simulink model "turbo_controller"  (R2025a)
settings: Solver=FixedStepAuto  StartTime=0.0  StopTime=inf  FixedStep=0.001  RelTol=1e-3
PostLoadFcn:
  | % 自动定位同目录CubeMX文件；不需要外部初始化脚本。
  | codertarget.data.setParameterValue('turbo_controller','STM32CubeMX.ProjectFile',fullfile(fileparts(get_param('turbo_controller','FileName')),'turbo_f407.ioc'));
InitFcn:
  | % 中文说明：按原控制器字段与类型创建三组接口总线；控制参数已内嵌。
  | tc_names=["EValve_Cycle" "EValve_Open" "Eblast_Cycle" "Eblast_Open" "Motor_Cycle" "Motor_Open" "EValve_Enable" "Eblast_Enable" "Motor_Enable" "SWO_Firework" "SWO_BleedAir" "EngineState" "Flag_ECUReset_Clear" "Flag_ECUReset_Save" "Flag_Reset_Enable" "Accelerator" "Nc_dem" "Nc"]; tc_types=["uint16" "uint16" "uint16" "uint16" "uint16" "uint16" "uint8" "uint8" "uint8" "uint8" "uint8" "uint8" "uint8" "uint8" "uint8" "single" "single" "single"];
  | for tc_k=1:numel(tc_names)
  |  tc_e(tc_k)=Simulink.BusElement; tc_e(tc_k).Name=char(tc_names(tc_k)); tc_e(tc_k).DataType=char(tc_types(tc_k));
  | end
  | EngineControl_Out=Simulink.Bus; EngineControl_Out.DataScope='Exported'; EngineControl_Out.Elements=tc_e;
  | clear tc_e tc_names tc_types tc_k
  | tc_names=["savedata1" "savedata2" "savedata3" "savedata4" "savedata5" "savedata6" "savedata7" "savedata8" "savedata9" "savedata10" "savedata11" "savedata12" "savedata13" "savedata14" "savedata15" "savedata16" "savedata17" "savedata18" "savedata19" "savedata20" "savedata21" "savedata22" "savedata23" "savedata24" "savedata25"]; tc_types=["single" "single" "single" "single" "single" "single" "single" "single" "single" "single" "single" "single" "single" "single" "single" "single" "single" "single" "single" "single" "single" "single" "single" "single" "single"];
  | for tc_k=1:numel(tc_names)
  |  tc_e(tc_k)=Simulink.BusElement; tc_e(tc_k).Name=char(tc_names(tc_k)); tc_e(tc_k).DataType=char(tc_types(tc_k));
  | end
  | SaveData_Out=Simulink.Bus; SaveData_Out.DataScope='Exported'; SaveData_Out.Elements=tc_e;
  | clear tc_e tc_names tc_types tc_k
  | tc_names=["senddata1" "senddata2" "senddata3" "senddata4" "senddata5" "senddata6" "senddata7" "senddata8" "senddata9" "senddata10" "senddata11" "senddata12" "senddata13" "senddata14" "senddata15" "senddata16" "senddata17" "senddata18" "senddata19" "senddata20" "senddata21" "senddata22" "senddata23" "senddata24" "senddata25" "senddata26" "senddata27" "senddata28" "senddata29"]; tc_types=["uint8" "uint8" "uint8" "uint8" "uint8" "uint8" "uint8" "uint8" "uint8" "uint8" "uint8" "uint8" "uint8" "uint8" "uint8" "uint8" "uint8" "uint8" "uint8" "uint8" "uint8" "uint8" "uint8" "uint8" "uint8" "uint8" "uint8" "uint8" "uint8"];
  | for tc_k=1:numel(tc_names)
  |  tc_e(tc_k)=Simulink.BusElement; tc_e(tc_k).Name=char(tc_names(tc_k)); tc_e(tc_k).DataType=char(tc_types(tc_k));
  | end
  | SendData_Out=Simulink.Bus; SendData_Out.DataScope='Exported'; SendData_Out.Elements=tc_e;
  | clear tc_e tc_names tc_types tc_k
  | 
  | % 以下为接口中文说明；只设置描述，不改变数值或数据类型。
  | EngineControl_Out.Description='执行控制输出（阀、电机、点火、状态及复位请求）';
  | tc_cn=["EValve_Cycle（主油阀周期计数（每计数2毫秒））" "EValve_Open（主油阀开通计数（每计数2毫秒））" "Eblast_Cycle（副油阀周期计数（每计数2毫秒））" "Eblast_Open（副油阀开通计数（每计数2毫秒））" "Motor_Cycle（起动电机周期计数）" "Motor_Open（起动电机开通计数）" "EValve_Enable（主油阀驱动使能）" "Eblast_Enable（副油阀驱动使能）" "Motor_Enable（起动电机使能）" "SWO_Firework（点火器使能（1开））" "SWO_BleedAir（引气阀使能（1开））" "EngineState（发动机状态）" "Flag_ECUReset_Clear（清除复位恢复状态请求）" "Flag_ECUReset_Save（保存复位恢复数据请求）" "Flag_Reset_Enable（处理器软件复位请求）" "Accelerator（油门／油泵给定控制量）" "Nc_dem（控制目标转速）" "Nc（发动机反馈转速（转每分））"];
  | tc_elements=EngineControl_Out.Elements;
  | for tc_k=1:numel(tc_cn)
  |  tc_elements(tc_k).Description=char(tc_cn(tc_k));
  | end
  | EngineControl_Out.Elements=tc_elements;
  | clear tc_cn tc_elements tc_k
  | SaveData_Out.Description='25项运行记录；字段含义按当前模型数据来源解释';
  | tc_cn=["savedata1（指令回显记录）" "savedata2（入口总温记录（℃））" "savedata3（电源电压记录）" "savedata4（排气温度记录（℃））" "savedata5（标定燃油压力记录）" "savedata6（副油阀占空比记录（％））" "savedata7（主油阀占空比记录（％））" "savedata8（温度修正转速记录）" "savedata9（开关输出及反馈位域）" "savedata10（物理转速记录）" "savedata11（油泵目标给定原始值）" "savedata12（起动电机占空比记录（％））" "savedata13（发动机状态码记录）" "savedata14（故障告警位域记录）" "savedata15（模型记录帧序号）" "savedata16（处理器温度记录（℃））" "savedata17（装订转速记录（沿用旧电源字段名））" "savedata18（导航高度记录）" "savedata19（飞行空速记录）" "savedata20（主阀旧记录位（恒零保留））" "savedata21（第21项保留记录（恒零））" "savedata22（保留记录项22）" "savedata23（保留记录项23）" "savedata24（保留记录项24）" "savedata25（保留记录项25）"];
  | tc_elements=SaveData_Out.Elements;
  | for tc_k=1:numel(tc_cn)
  |  tc_elements(tc_k).Description=char(tc_cn(tc_k));
  | end
  | SaveData_Out.Elements=tc_elements;
  | clear tc_cn tc_elements tc_k
  | SendData_Out.Description='29字段回传及外设命令接口；板端上位机帧只取第3至27字段';
  | tc_cn=["senddata1（回传发送允许标志（不直接上线路））" "senddata2（回传载荷长度25字节）" "senddata3（回传指令回显字节）" "senddata4（总温编码字节（℃＋80））" "senddata5（电源电压编码字节）" "senddata6（排温编码高字节）" "senddata7（排温编码低字节）" "senddata8（燃油压力编码高字节）" "senddata9（燃油压力编码低字节）" "senddata10（副油阀占空比字节（％））" "senddata11（主油阀占空比字节（％））" "senddata12（修正转速编码高字节）" "senddata13（修正转速编码低字节）" "senddata14（驱动及反馈状态位域）" "senddata15（物理转速编码高字节）" "senddata16（物理转速编码低字节）" "senddata17（油泵目标给定高字节（串口二使用））" "senddata18（油泵目标给定低字节（串口二使用））" "senddata19（起动电机占空比命令（串口一使用））" "senddata20（发动机状态码字节）" "senddata21（故障告警位域字节）" "senddata22（帧序号占位（板端另行填写））" "senddata23（处理器温度编码（℃＋50））" "senddata24（控制目标转速编码高字节）" "senddata25（控制目标转速编码低字节）" "senddata26（占位字节（板端改填实测泵速高字节））" "senddata27（占位字节（板端改填实测泵速低字节））" "senddata28（装订转速高字节（本板未发送））" "senddata29（装订转速低字节（本板未发送））"];
  | tc_elements=SendData_Out.Elements;
  | for tc_k=1:numel(tc_cn)
  |  tc_elements(tc_k).Description=char(tc_cn(tc_k));
  | end
  | SendData_Out.Elements=tc_elements;
  | clear tc_cn tc_elements tc_k
  | 
  | 
  | % FRAM模块化事务：接口类型和上电初始状态，随模型保存，无外部初始化文件。
  | clear FM_elements
  | FM_elements(1)=Simulink.BusElement;FM_elements(1).Name='phase';FM_elements(1).DataType='uint8';FM_elements(1).Dimensions=[1 1];FM_elements(1).Description='phase（当前事务阶段）';
  | FM_elements(2)=Simulink.BusElement;FM_elements(2).Name='a';FM_elements(2).DataType='uint8';FM_elements(2).Dimensions=[64 1];FM_elements(2).Description='a（启动时缓存的首区64字节）';
  | FM_elements(3)=Simulink.BusElement;FM_elements(3).Name='active';FM_elements(3).DataType='uint16';FM_elements(3).Dimensions=[1 1];FM_elements(3).Description='active（当前有效记录区地址）';
  | FM_elements(4)=Simulink.BusElement;FM_elements(4).Name='generation';FM_elements(4).DataType='uint32';FM_elements(4).Dimensions=[1 1];FM_elements(4).Description='generation（当前有效记录代号）';
  | FM_elements(5)=Simulink.BusElement;FM_elements(5).Name='record';FM_elements(5).DataType='uint8';FM_elements(5).Dimensions=[64 1];FM_elements(5).Description='record（本次冻结的待写记录）';
  | FM_elements(6)=Simulink.BusElement;FM_elements(6).Name='addr';FM_elements(6).DataType='uint16';FM_elements(6).Dimensions=[1 1];FM_elements(6).Description='addr（本次备用写入地址）';
  | FM_elements(7)=Simulink.BusElement;FM_elements(7).Name='lastSave';FM_elements(7).DataType='single';FM_elements(7).Dimensions=[1 1];FM_elements(7).Description='lastSave（上次开始保存的秒数）';
  | FM_elements(8)=Simulink.BusElement;FM_elements(8).Name='lastState';FM_elements(8).DataType='uint8';FM_elements(8).Dimensions=[1 1];FM_elements(8).Description='lastState（上次保存时的发动机状态）';
  | FM_elements(9)=Simulink.BusElement;FM_elements(9).Name='boot';FM_elements(9).DataType='boolean';FM_elements(9).Dimensions=[1 1];FM_elements(9).Description='boot（启动记录是否允许恢复）';
  | FM_elements(10)=Simulink.BusElement;FM_elements(10).Name='consumed';FM_elements(10).DataType='boolean';FM_elements(10).Dimensions=[1 1];FM_elements(10).Description='consumed（本次启动恢复通知是否已发送）';
  | FM_elements(11)=Simulink.BusElement;FM_elements(11).Name='payload';FM_elements(11).DataType='uint8';FM_elements(11).Dimensions=[20 1];FM_elements(11).Description='payload（当前20字节恢复内容）';
  | ... (+35 lines)
model workspace (MAT data in the model file):
  CRC16_Table_Reference = [0 4129 8258 12387 16516 20645 24774 28903 33032 37161 41290 45419 ... (256 elements, 256x1)]
  PE_Kaer = [0.15402 0.15402 0.12264 0.10076 0.09481 0.07601 0.07111 0.0569 0.05198 0.04926 0.05308 0.04325 ... (13 elements, 1x13)]
  PE_Nr = [21.2982 61.4260372 67.7475458 72.7394382 76.845934 80.6988798 83.8449282 86.6491912 88.9382406 89.178606 91.1938214 93.4068058 ... (13 elements, 1x13)]
  PE_Pump_Translate = 33.5999984741
  PE_RotaSpeed_Translate = 860
  PE_Taer = [0.4939154 0.4939154 0.40780982 0.34066978 0.31622756 0.30405716 0.34300244 0.26785022 0.37393554 0.23914836 0.44563948 0.31044662 ... (13 elements, 1x13)]
  PF_ACCFULLRANGE = 3360
  PF_Flag_ECUReset = 0
  PF_Flag_rx_suc = 1
  PF_Gear_Info = [40000; 45000; 50000; 55000; 57000; 59000; 60000; 61000; 61000; 61000; 61000; 61000]
  PF_K_TiaoJie = 1
  PF_Kpu = 10
  PF_MySet_Rxdata = [0 0 0 0 0 0 0 0 0 0 0 0 ... (50 elements, 50x1)]
  PF_MyUsart1_Rxdata = [0 0 0 0 0 0 0 0 0 0 0 0 ... (50 elements, 50x1)]
  PF_MyUsart2_Rxdata = [0 0 0 0 0 0 0 0 0 0 0 0 ... (50 elements, 50x1)]
  PF_Reset_Information = [0 0 0 0 0 0 0 0 0 0 0 0 ... (20 elements, 20x1)]
  PF_Sensor_X1_T4 = [0 4095]
  PF_Sensor_X2_T4 = [0 1.66666698456]
  PF_Sensor_X3_T4 = [0 504 999 1497 2010 2529 3051 3568 4076 4571 4959]
  PF_Sensor_X_P2 = [0.5 3]
  PF_Sensor_X_Poil = [0.5 3]
  PF_Sensor_X_T1t = [-50 300]
  PF_Sensor_X_Vpower = [0 3]
  PF_Sensor_X_Vpump = [0 3]
  PF_Sensor_Y1_T4 = [0 3]
  PF_Sensor_Y2_T4 = [0 5000]
  PF_Sensor_Y3_T4 = [0 100 200 300 400 500 600 700 800 900 980]
  PF_Sensor_Y_P2 = [0 1000]
  PF_Sensor_Y_Poil = [0 1000]
  PF_Sensor_Y_T1t = [-50 300]
  PF_Sensor_Y_Vpower = [0 33]
  PF_Sensor_Y_Vpump = [0 33]
  PG_CtrlMode_CloseLoop : mpt.Parameter (value not decoded)
  PG_CtrlMode_ManualAcc : mpt.Parameter (value not decoded)
  PG_CtrlMode_Origin : mpt.Parameter (value not decoded)
  PG_CtrlMode_Start : mpt.Parameter (value not decoded)
  PG_CtrlMode_Stop : mpt.Parameter (value not decoded)
  PG_ES_Clp : mpt.Parameter (value not decoded)
  PG_ES_EngStart : mpt.Parameter (value not decoded)
  PG_ES_Manual : mpt.Parameter (value not decoded)
  PG_ES_Origin : mpt.Parameter (value not decoded)
  PG_ES_Stop : mpt.Parameter (value not decoded)
  PG_Instr_BleedAirSet : mpt.Parameter (value not decoded)
  PG_Instr_CloseLoop : mpt.Parameter (value not decoded)
  PG_Instr_ECUReSet : mpt.Parameter (value not decoded)
  PG_Instr_EValveSet : mpt.Parameter (value not decoded)
  PG_Instr_EblastSet : mpt.Parameter (value not decoded)
  PG_Instr_Erase : mpt.Parameter (value not decoded)
  PG_Instr_FireWorkSet : mpt.Parameter (value not decoded)
  PG_Instr_ManualPlus : mpt.Parameter (value not decoded)
  PG_Instr_ManualrReduce : mpt.Parameter (value not decoded)
  PG_Instr_MotorSet : mpt.Parameter (value not decoded)
  PG_Instr_OilSet : mpt.Parameter (value not decoded)
  PG_Instr_SelfCheck : mpt.Parameter (value not decoded)
  PG_Instr_Start : mpt.Parameter (value not decoded)
  PG_Instr_Stop : mpt.Parameter (value not decoded)
  PG_Instr_StopZero : Simulink.Parameter (value not decoded)
  PG_Location_Air : Simulink.Parameter (value not decoded)
  PG_Location_Gnd : Simulink.Parameter (value not decoded)
  PG_ServoCtrlMode_CloseLoop : Simulink.Parameter (value not decoded)
  PG_ServoCtrlMode_CloseLoopMax : Simulink.Parameter (value not decoded)
  PG_ServoCtrlMode_CloseLoopMin : Simulink.Parameter (value not decoded)
  PG_ServoCtrlMode_ManualAcc : Simulink.Parameter (value not decoded)
  PG_ServoCtrlMode_ManualAccMax : Simulink.Parameter (value not decoded)
  PG_ServoCtrlMode_ManualAccMin : Simulink.Parameter (value not decoded)
  PG_SpeedDot_Permit : Simulink.Parameter (value not decoded)
  PL_EngineModel_Actuator = [0 10 100]
  PL_EngineModel_EngineStar_Press_P2 = [1013 1098.4 1099.144828 1099.931034 1103.613793 1162.662069 1143.793103 1131.006897 1123.186207 1117.6 1114 1111.806897 ... (127 elements, 1x127)]
  PL_EngineModel_EngineStar_RotaSpeed = [200 2000 9584 9660 10220 10240 10260 10288 10308 10368 10380 10408 ... (127 elements, 1x127)]
  PL_EngineModel_EngineStar_Temp_Exhaust = [128 129 129.1 130 131 131.1 132 133 134 134.1 135 135.1 ... (127 elements, 1x127)]
  PL_EngineModel_EngineStar_Time = [0.05 0.1 0.15 0.2 0.25 0.3 0.35 0.4 0.45 0.5 0.55 0.6 ... (127 elements, 1x127)]
  PL_EngineModel_IdleAbove_Nr = [0 21.2982 61.4260372 67.7475458 72.7394382 76.845934 80.6988798 83.8449282 86.6491912 88.9382406 89.178606 91.1938214 ... (14 elements, 1x14)]
  PL_EngineModel_IdleAbove_P2r = [0.986923266716 1.57907722675 1.81593881076 1.99358499877 2.23044658278 2.43770046879 2.65482358747 2.84233900814 3.03972366149 3.18776215149 3.25684678016 3.3950160375 ... (14 elements, 1x14)]
  PL_EngineModel_IdleAbove_Tempr = [0.0536001429337 1.07200285867 1.63301768805 1.63659103091 1.66875111667 1.72592460247 1.77595140254 1.86171163123 1.95461854565 2.03323208862 2.03323208862 2.13685903162 ... (14 elements, 1x14)]
  PL_EngineModel_IdleAbove_Ter = [0.42434128 0.42434128 0.42434128 0.30669408 0.23570008 0.22150128 0.1997974 0.23803274 0.16115638 0.24279948 0.13600422 0.31308354 ... (14 elements, 1x14)]
  PL_EngineModel_IdleAbove_Wfr = [0 10.142 23.8337 27.8905 31.9473 36.0041 40.0609 44.1177 48.1745 52.2313 52.7384 56.7952 ... (14 elements, 1x14)]
  PL_EngineModel_Press_P2 = [400 400 400 400 400 400 400 400 400 400]
  PL_EngineModel_Rotaspeed = [0 20000 96400]
  PL_EngineModel_Temp_Exhaust = [500 500 500 500 500 500 500 500 500 500]
  PL_Kaer = [0.1 0.1 0.1 0.1 0.1 0.1]
  PL_Nr = [50 60 70 80 90 100]
  PL_Taer = [0.1 0.1 0.1 0.1 0.1 0.1]
  Sig : Simulink.Signal (value not decoded)
  Ts_ms : Simulink.Parameter (value not decoded)
  false : Simulink.Parameter (value not decoded)
  true : Simulink.Parameter (value not decoded)
symbols that are objects in the model workspace (value not decoded): PG_CtrlMode_CloseLoop, PG_CtrlMode_ManualAcc, PG_CtrlMode_Origin, PG_CtrlMode_Start, PG_CtrlMode_Stop, PG_ES_Clp, PG_ES_EngStart, PG_ES_Manual, PG_ES_Origin, PG_ES_Stop, PG_Instr_BleedAirSet, PG_Instr_CloseLoop, PG_Instr_EblastSet, PG_Instr_ECUReSet, PG_Instr_Erase, PG_Instr_EValveSet, PG_Instr_FireWorkSet, PG_Instr_ManualPlus, PG_Instr_ManualrReduce, PG_Instr_MotorSet, PG_Instr_OilSet, PG_Instr_SelfCheck, PG_Instr_Start, PG_Instr_Stop, PG_Instr_StopZero, PG_ServoCtrlMode_CloseLoop, PG_ServoCtrlMode_CloseLoopMax, PG_ServoCtrlMode_CloseLoopMin, PG_ServoCtrlMode_ManualAcc, PG_ServoCtrlMode_ManualAccMax, PG_ServoCtrlMode_ManualAccMin, Ts_ms
libraries: simulink x97, stm32blockslib x10, stm32f4xxblockslib x8
(part 12 of 26)

== system turbo_controller/BoardOutput_串口封装与阀门时序/Out02_Timing（阀门与点火时序）/MainValve（主阀周期与开度）_719 ==
  note: 主阀怎样按周期形成开启区间
      |
      | 本模块收到使能Enable、周期计数Cycle、开启计数Open，以及父级给出的偶数毫秒节拍Even。它输出
      | 的是逻辑开启状态On，父级随后才按低有效电路把它取反成引脚电平。
      |
      | 先检查Enable是否非零、Cycle是否非零，两者都成立才允许运行。对Cycle为零的情况，SafeCycle提
      | 供1作为取余用的安全分母，但运行许可仍为假，所以不会因为避免除零而误开阀。
      |
      | 内部Phase记住周期位置，在2 ms节拍内按先归一化、后推进的分支更新。位置到周期末尾通过取余回
      | 到起点；位置小于Open时On为真，其余区间为假。
      |
      | 例如Cycle=30、Open=15，约每60 ms重复一次，其中约30 ms开启；Open=0则没有开启区间，Open不小
      | 于周期时允许区间覆盖整个周期。这里的15是15个2 ms计数，不是15 ms。
      |
      | 禁止使能时按关闭支路处理，不能仅看历史Phase猜测当前输出。位置跨1 ms调用保存，是周期波形成
      | 立所必需的状态。
  Enable（阀门使能）_692 : Inport
  Cycle（周期计数）_693 : Inport  Port=2
  Open（开启计数）_695 : Inport  Port=3
  Even（本毫秒为偶数节拍）_697 : Inport  Port=4  OutDataTypeStr=boolean
  Add（加减运算）_716 : Sum  SaturateOnIntegerOverflow=on  OutDataTypeStr=Inherit: Same as first input
  Advance（奇数毫秒推进一次计数）_717 : Switch  Criteria=u2 ~= 0  SaturateOnIntegerOverflow=off  InputSameDT=off
  Cast（数据类型转换）_694 : DataTypeConversion  OutDataTypeStr=uint32  RndMeth=Round
  Cast（数据类型转换）_696 : DataTypeConversion  OutDataTypeStr=uint32  RndMeth=Round
  Cast（数据类型转换）_706 : DataTypeConversion  OutDataTypeStr=double  RndMeth=Round
  Cast（数据类型转换）_707 : DataTypeConversion  OutDataTypeStr=double  RndMeth=Round
  Cast（数据类型转换）_709 : DataTypeConversion  OutDataTypeStr=uint32  RndMeth=Floor
  Constant（常量）_699 : Constant  Value=0  OutDataTypeStr=uint8
  Constant（常量）_701 : Constant  Value=0  OutDataTypeStr=uint32
  Constant（常量）_704 : Constant  OutDataTypeStr=uint32
  Constant（常量）_710 : Constant  Value=0  OutDataTypeStr=uint32
  Constant（常量）_715 : Constant  OutDataTypeStr=uint32
  CycleValid（周期不为零）_702 : RelationalOperator  Operator=~=  OutDataTypeStr=boolean  RndMeth=Simplest  InputSameDT=off
  Enabled（使能不为零）_700 : RelationalOperator  Operator=~=  OutDataTypeStr=boolean  RndMeth=Simplest  InputSameDT=off
  InsideOpen（当前位于开启区间）_713 : RelationalOperator  Operator=<  OutDataTypeStr=boolean  RndMeth=Simplest  InputSameDT=off
  Phase（跨毫秒保存的周期位置）_698 : UnitDelay  InitialCondition=uint32(0)  SampleTime=-1  HasFrameUpgradeWarning=on
  Running（允许周期运行）_703 : Logic  IconShape=distinctive  AllPortsSameDT=off  OutDataTypeStr=boolean
  SafeCycle（零周期时避免取余异常）_705 : Switch  Criteria=u2 ~= 0  SaturateOnIntegerOverflow=off  InputSameDT=off
  Select（按条件选择）_711 : Switch  Criteria=u2 ~= 0  SaturateOnIntegerOverflow=off  InputSameDT=off
  Store_uint32（按三十二位无符号数保存状态）_537181 : DataTypeConversion  Description=为反馈回路显式指定原程序的状态类型，保持原状态更新节拍。  OutDataTypeStr=uint32  RndMeth=Round
  Update2ms（每两毫秒归一化周期位置）_712 : Switch  Criteria=u2 ~= 0  SaturateOnIntegerOverflow=off  InputSameDT=off
  ValveOn（本毫秒阀门开启）_714 : Logic  IconShape=distinctive  AllPortsSameDT=off  OutDataTypeStr=boolean
  WrapCycle（按周期长度回卷）_708 : Math  Operator=mod
  On（逻辑开启状态）_718 : Outport
  wires:
  Constant（常量）_701/1 -> CycleValid（周期不为零）_702/2  "Constant（常量）"
  Cast（数据类型转换）_694/1 -> CycleValid（周期不为零）_702/1, SafeCycle（零周期时避免取余异常）_705/1  "Cast（数据类型转换）"
  Cycle（周期计数）_693/1 -> Cast（数据类型转换）_694/1  "Cycle（周期计数）"
  Constant（常量）_704/1 -> SafeCycle（零周期时避免取余异常）_705/3  "Constant（常量）"
  CycleValid（周期不为零）_702/1 -> SafeCycle（零周期时避免取余异常）_705/2, Running（允许周期运行）_703/2  "CycleValid（周期不为零）"
  SafeCycle（零周期时避免取余异常）_705/1 -> Cast（数据类型转换）_707/1  "SafeCycle（零周期时避免取余异常）"
  Enable（阀门使能）_692/1 -> Enabled（使能不为零）_700/1  "Enable（阀门使能）"
  Cast（数据类型转换）_707/1 -> WrapCycle（按周期长度回卷）_708/2  "Cast（数据类型转换）"
  Constant（常量）_699/1 -> Enabled（使能不为零）_700/2  "Constant（常量）"
  WrapCycle（按周期长度回卷）_708/1 -> Cast（数据类型转换）_709/1  "WrapCycle（按周期长度回卷）"
  Enabled（使能不为零）_700/1 -> Running（允许周期运行）_703/1  "Enabled（使能不为零）"
  Cast（数据类型转换）_709/1 -> Select（按条件选择）_711/1  "Cast（数据类型转换）"
  Running（允许周期运行）_703/1 -> Select（按条件选择）_711/2, ValveOn（本毫秒阀门开启）_714/1  "Running（允许周期运行）"
  Constant（常量）_710/1 -> Select（按条件选择）_711/3  "Constant（常量）"
  Open（开启计数）_695/1 -> Cast（数据类型转换）_696/1  "Open（开启计数）"
  Select（按条件选择）_711/1 -> Update2ms（每两毫秒归一化周期位置）_712/1  "Select（按条件选择）"
  Even（本毫秒为偶数节拍）_697/1 -> Update2ms（每两毫秒归一化周期位置）_712/2, Advance（奇数毫秒推进一次计数）_717/2  "Even（本毫秒为偶数节拍）"
  Cast（数据类型转换）_696/1 -> InsideOpen（当前位于开启区间）_713/2  "Cast（数据类型转换）"
  Update2ms（每两毫秒归一化周期位置）_712/1 -> Advance（奇数毫秒推进一次计数）_717/1, Add（加减运算）_716/1, InsideOpen（当前位于开启区间）_713/1  "Update2ms（每两毫秒归一化周期位置）"
  Constant（常量）_715/1 -> Add（加减运算）_716/2  "Constant（常量）"
  InsideOpen（当前位于开启区间）_713/1 -> ValveOn（本毫秒阀门开启）_714/2  "InsideOpen（当前位于开启区间）"
  Add（加减运算）_716/1 -> Advance（奇数毫秒推进一次计数）_717/3  "Add（加减运算）"
  ValveOn（本毫秒阀门开启）_714/1 -> On（逻辑开启状态）_718/1  "ValveOn（本毫秒阀门开启）"
  Advance（奇数毫秒推进一次计数）_717/1 -> Store_uint32（按三十二位无符号数保存状态）_537181/1  "Advance（奇数毫秒推进一次计数）"
  Store_uint32（按三十二位无符号数保存状态）_537181/1 -> Phase（跨毫秒保存的周期位置）_698/1
  Phase（跨毫秒保存的周期位置）_698/1 -> Update2ms（每两毫秒归一化周期位置）_712/3, Cast（数据类型转换）_706/1  "Phase（跨毫秒保存的周期位置）"
  Cast（数据类型转换）_706/1 -> WrapCycle（按周期长度回卷）_708/1  "Cast（数据类型转换）"

== system turbo_controller/BoardOutput_串口封装与阀门时序/Out03_Telemetry（上位机回传组帧）/Checksum（累加与异或校验）_211 ==
  note: 一段字节怎样得到累加和异或两种校验
      |
      | 输入是一整段需要校验的字节。每帧开始，两路累积值都从0开始；For Iterator按顺序取出每个字节
      | ，同时更新两路结果。
      |
      | 累加这一路只保留低8位：
      | 新累加值 = mod(旧累加值 + 当前字节,256)。
      | 例如三个字节为200、100、1，总和301，最后校验字节为45，不让普通uint8溢出替代明确的取余规则
      | 。
      |
      | 异或这一路逐位计算：
      | 新异或值 = bitxor(旧异或值,当前字节)。
      | 相同比特异或得到0，不同比特得到1。它与“所有数相加”是两种不同检查。
      |
      | 接收侧拿这两个结果和帧尾比较，发送侧把结果追加到帧尾。父级负责规定哪些字节参加计算；本模块
      | 不验证帧头，也不能替换电机/油泵协议使用的CRC16。
  Bytes（待校验字节）_196 : Inport  OutDataTypeStr=uint8
  Add（加减运算）_203 : Sum  SaturateOnIntegerOverflow=on  OutDataTypeStr=Inherit: Same as first input
  Cast（数据类型转换）_201 : DataTypeConversion  OutDataTypeStr=double  RndMeth=Round
  Cast（数据类型转换）_202 : DataTypeConversion  OutDataTypeStr=double  RndMeth=Round
  Cast（数据类型转换）_206 : DataTypeConversion  OutDataTypeStr=uint8  RndMeth=Floor
  Constant（常量）_204 : Constant  Value=256  OutDataTypeStr=double
  EachByte（逐字节累加与异或）_197 : ForIterator  ResetStates=reset  IterationLimit=28  IterationVariableDataType=uint32
  Select（按索引取元素）_200 : Selector  InputPortWidth=28  IndexOptions=Index vector (port)  Indices=1  OutputSizes=1
  Store（保持原状态类型）_208 : DataTypeConversion  OutDataTypeStr=uint8  RndMeth=Round
  Sum（本帧累加器）_198 : UnitDelay  InitialCondition=uint8(0)  SampleTime=-1  HasFrameUpgradeWarning=on
  Wrap8（累加后只保留八位）_205 : Math  Operator=mod
  XorStep（异或一个字节）_207 : simulink/Logic and Bit Operations/Bitwise Operator  logicop=XOR  UseBitMask=off  NumInputPorts=2  BitMask=bin2dec('11011001')  BitMaskRealWorld=Stored Integer
      settings: LibrarySourceBlock=|
      | hdlsllib/Logic and Bit
      | Operations/Bitwise
      | Operator
  Xor（本帧异或器）_199 : UnitDelay  InitialCondition=uint8(0)  SampleTime=-1  HasFrameUpgradeWarning=on
  Sum8（八位累加结果）_209 : Outport
  Xor8（八位异或结果）_210 : Outport  Port=2
  wires:
  Store（保持原状态类型）_208/1 -> Xor（本帧异或器）_199/1  "Store（保持原状态类型）"
  XorStep（异或一个字节）_207/1 -> Xor8（八位异或结果）_210/1, Store（保持原状态类型）_208/1  "XorStep（异或一个字节）"
  Cast（数据类型转换）_206/1 -> Sum8（八位累加结果）_209/1, Sum（本帧累加器）_198/1  "Cast（数据类型转换）"
  Xor（本帧异或器）_199/1 -> XorStep（异或一个字节）_207/1  "Xor（本帧异或器）"
  Wrap8（累加后只保留八位）_205/1 -> Cast（数据类型转换）_206/1  "Wrap8（累加后只保留八位）"
  Constant（常量）_204/1 -> Wrap8（累加后只保留八位）_205/2  "Constant（常量）"
  Add（加减运算）_203/1 -> Wrap8（累加后只保留八位）_205/1  "Add（加减运算）"
  Cast（数据类型转换）_202/1 -> Add（加减运算）_203/2  "Cast（数据类型转换）"
  Cast（数据类型转换）_201/1 -> Add（加减运算）_203/1  "Cast（数据类型转换）"
  Select（按索引取元素）_200/1 -> XorStep（异或一个字节）_207/2, Cast（数据类型转换）_202/1  "Select（按索引取元素）"
  Sum（本帧累加器）_198/1 -> Cast（数据类型转换）_201/1  "Sum（本帧累加器）"
  EachByte（逐字节累加与异或）_197/1 -> Select（按索引取元素）_200/2  "EachByte（逐字节累加与异或）"
  Bytes（待校验字节）_196/1 -> Select（按索引取元素）_200/1  "Bytes（待校验字节）"

== system turbo_controller/BoardOutput_串口封装与阀门时序/Out03_Telemetry（上位机回传组帧）/Clock20ms（二十毫秒通信节拍）_126 ==
  note: 从秒数产生每二十毫秒一次的许可
      |
      | 本模块收到当前模型时间Seconds。先乘1000换成毫秒，再对20取余，判断余数是否小于1：
      | 工作许可 = mod(Seconds×1000,20)<1。
      |
      | 在父级1 ms离散调用下，约在0、20、40、60 ms等时刻为真，中间毫秒为假。用“小于1”表示当前1 m
      | s时间格，避免把它理解成连续时间的一次精确相等判断。
      |
      | 这只是一个布尔许可，不会让模型等待或暂停。转速选择用它决定何时更新Speed，回传组帧用它决定
      | 何时生成新帧；其他1 ms任务继续正常运行。
  Seconds（当前秒数）_117 : Inport  OutDataTypeStr=double
  Constant（常量）_118 : Constant  Value=1000  OutDataTypeStr=double
  Constant（常量）_121 : Constant  Value=20  OutDataTypeStr=double
  Constant（常量）_123 : Constant  Value=0  OutDataTypeStr=double
  Every20ms（20毫秒更新许可）_124 : RelationalOperator  Operator===  OutDataTypeStr=boolean  RndMeth=Simplest  InputSameDT=off
  Milliseconds（秒换算为毫秒）_119 : Product  Inputs=**  SaturateOnIntegerOverflow=on  OutDataTypeStr=Inherit: Same as first input
  Phase20（20毫秒相位）_122 : Math  Operator=mod
  RoundTime（按原规则取整）_120 : Rounding  Operator=round
  Every20ms（二十毫秒更新许可）_125 : Outport
  wires:
  Every20ms（20毫秒更新许可）_124/1 -> Every20ms（二十毫秒更新许可）_125/1  "Every20ms（20毫秒更新许可）"
  Constant（常量）_123/1 -> Every20ms（20毫秒更新许可）_124/2  "Constant（常量）"
  Phase20（20毫秒相位）_122/1 -> Every20ms（20毫秒更新许可）_124/1  "Phase20（20毫秒相位）"
  Constant（常量）_121/1 -> Phase20（20毫秒相位）_122/2  "Constant（常量）"
  RoundTime（按原规则取整）_120/1 -> Phase20（20毫秒相位）_122/1  "RoundTime（按原规则取整）"
  Milliseconds（秒换算为毫秒）_119/1 -> RoundTime（按原规则取整）_120/1  "Milliseconds（秒换算为毫秒）"
  Constant（常量）_118/1 -> Milliseconds（秒换算为毫秒）_119/2  "Constant（常量）"
  Seconds（当前秒数）_117/1 -> Milliseconds（秒换算为毫秒）_119/1  "Seconds（当前秒数）"

== system turbo_controller/BoardOutput_串口封装与阀门时序/Out03_Telemetry（上位机回传组帧）/FrameCounter（循环帧号）_138 ==
  note: 用循环帧号辨认相邻回传帧
      |
      | 输入Tick表示本次是否到20 ms通信更新时刻。内部记忆块保存上一帧号，本模块在Tick有效时加1，达
      | 到字节上限后回到0；Tick无效时保持。
      |
      | 更新规律可理解为下一帧号=mod(旧帧号+1,256)。例如旧值254，下一次255，再下一次0，而不是让uin
      | t8相加后出现未说明的溢出。
      |
      | 帧号交给Payload，覆盖最终28字节内容中的第23项，帮助上位机观察帧的先后和是否漏接。它不是发
      | 动机状态、转速，也不是已经运行的秒数。
  Control（二十毫秒更新许可）_127 : Inport  OutDataTypeStr=boolean
  Add（加减运算）_131 : Sum  SaturateOnIntegerOverflow=on  OutDataTypeStr=Inherit: Same as first input
  Cast（数据类型转换）_129 : DataTypeConversion  OutDataTypeStr=double  RndMeth=Round
  Cast（数据类型转换）_134 : DataTypeConversion  OutDataTypeStr=uint8  RndMeth=Floor
  Constant（常量）_130 : Constant  OutDataTypeStr=double
  Constant（常量）_132 : Constant  Value=256  OutDataTypeStr=double
  Counter（当前帧号）_128 : UnitDelay  InitialCondition=uint8(0)  SampleTime=-1  HasFrameUpgradeWarning=on
  Select（按条件选择）_135 : Switch  Criteria=u2 ~= 0  SaturateOnIntegerOverflow=off  InputSameDT=off
  StoreCounter（保存下一帧号）_136 : DataTypeConversion  OutDataTypeStr=uint8  RndMeth=Round
  Wrap（二百五十五之后回到零）_133 : Math  Operator=mod
  Counter（当前帧使用的帧号）_137 : Outport
  wires:
  StoreCounter（保存下一帧号）_136/1 -> Counter（当前帧号）_128/1  "StoreCounter（保存下一帧号）"
  Select（按条件选择）_135/1 -> StoreCounter（保存下一帧号）_136/1  "Select（按条件选择）"
  Control（二十毫秒更新许可）_127/1 -> Select（按条件选择）_135/2  "Control（二十毫秒更新许可）"
  Cast（数据类型转换）_134/1 -> Select（按条件选择）_135/1  "Cast（数据类型转换）"
  Wrap（二百五十五之后回到零）_133/1 -> Cast（数据类型转换）_134/1  "Wrap（二百五十五之后回到零）"
  Constant（常量）_132/1 -> Wrap（二百五十五之后回到零）_133/2  "Constant（常量）"
  Add（加减运算）_131/1 -> Wrap（二百五十五之后回到零）_133/1  "Add（加减运算）"
  Constant（常量）_130/1 -> Add（加减运算）_131/2  "Constant（常量）"
  Cast（数据类型转换）_129/1 -> Add（加减运算）_131/1  "Cast（数据类型转换）"
  Counter（当前帧号）_128/1 -> Cast（数据类型转换）_129/1, Counter（当前帧使用的帧号）_137/1, Select（按条件选择）_135/3  "Counter（当前帧号）"

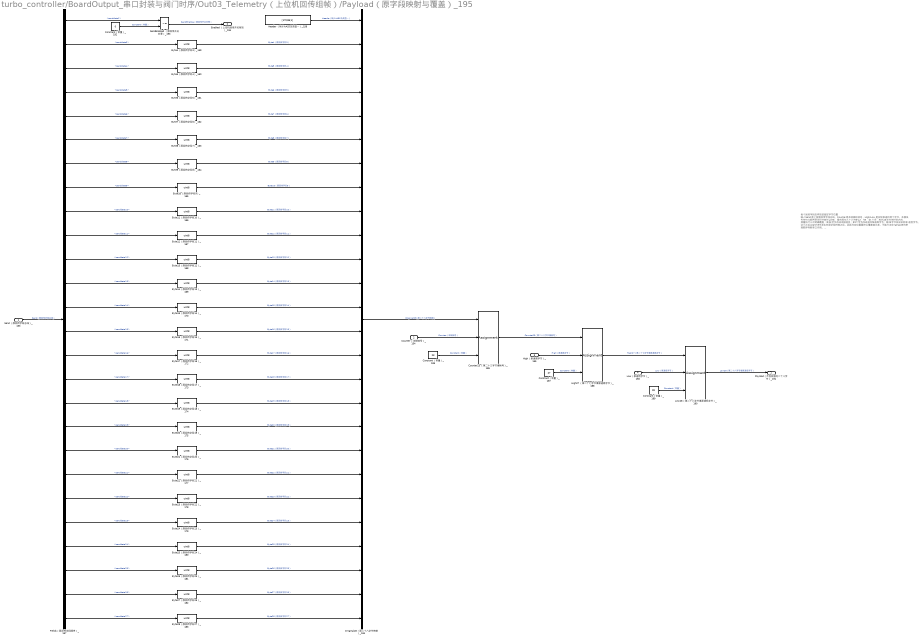
== system turbo_controller/BoardOutput_串口封装与阀门时序/Out03_Telemetry（上位机回传组帧）/Payload（原字段映射与覆盖）_195 ==
  note: 每个回传字段怎样放进固定字节位置
      |
      | 输入Send是上层原回传字段总线，Counter是本帧循环帧号，High/Low是实际泵速的两个字节。本模块
      | 先按协议顺序取字段并转成uint8，最前面加入十六进制AA、55、01三项，构成28字节待校验内容。
      |
      | 接着执行三次明确覆盖：第23字节改成本帧帧号；第27字节改成实际泵速高字节；第28字节改成实际泵
      | 速低字节。
      | 这三次Assignment发生在原字段拼接之后，因此对应位置最终以覆盖值为准，不能只读Original28的拼
      | 接顺序判断串口内容。
      |
      | 例如平滑泵速1000会以高3、低232进入第27/28字节；帧号从255回0时只改变第23项。SendEnabled另外
      | 判断原回传开关是否非零，它是发送许可，不占一个新的帧数据位置。
      |
      | 输出28字节交Checksum计算两项校验，父级再追加为30字节最终帧。本模块不直接启动UART。
  Send（原回传字段总线）_153 : Inport  OutDataTypeStr=Bus: SendData_Out
  Counter（本帧帧号）_154 : Inport  Port=2  OutDataTypeStr=uint8
  High（泵速高字节）_155 : Inport  Port=3  OutDataTypeStr=uint8
  Low（泵速低字节）_156 : Inport  Port=4  OutDataTypeStr=uint8
  Byte10（原回传字段9）_165 : DataTypeConversion  OutDataTypeStr=uint8  RndMeth=Round
  Byte11（原回传字段10）_166 : DataTypeConversion  OutDataTypeStr=uint8  RndMeth=Round
  Byte12（原回传字段11）_167 : DataTypeConversion  OutDataTypeStr=uint8  RndMeth=Round
  Byte13（原回传字段12）_168 : DataTypeConversion  OutDataTypeStr=uint8  RndMeth=Round
  Byte14（原回传字段13）_169 : DataTypeConversion  OutDataTypeStr=uint8  RndMeth=Round
  Byte15（原回传字段14）_170 : DataTypeConversion  OutDataTypeStr=uint8  RndMeth=Round
  Byte16（原回传字段15）_171 : DataTypeConversion  OutDataTypeStr=uint8  RndMeth=Round
  Byte17（原回传字段16）_172 : DataTypeConversion  OutDataTypeStr=uint8  RndMeth=Round
  Byte18（原回传字段17）_173 : DataTypeConversion  OutDataTypeStr=uint8  RndMeth=Round
  Byte19（原回传字段18）_174 : DataTypeConversion  OutDataTypeStr=uint8  RndMeth=Round
  Byte20（原回传字段19）_175 : DataTypeConversion  OutDataTypeStr=uint8  RndMeth=Round
  Byte21（原回传字段20）_176 : DataTypeConversion  OutDataTypeStr=uint8  RndMeth=Round
  Byte22（原回传字段21）_177 : DataTypeConversion  OutDataTypeStr=uint8  RndMeth=Round
  Byte23（原回传字段22）_178 : DataTypeConversion  OutDataTypeStr=uint8  RndMeth=Round
  Byte24（原回传字段23）_179 : DataTypeConversion  OutDataTypeStr=uint8  RndMeth=Round
  Byte25（原回传字段24）_180 : DataTypeConversion  OutDataTypeStr=uint8  RndMeth=Round
  Byte26（原回传字段25）_181 : DataTypeConversion  OutDataTypeStr=uint8  RndMeth=Round
  Byte27（原回传字段26）_182 : DataTypeConversion  OutDataTypeStr=uint8  RndMeth=Round
  Byte28（原回传字段27）_183 : DataTypeConversion  OutDataTypeStr=uint8  RndMeth=Round
  Byte4（原回传字段3）_159 : DataTypeConversion  OutDataTypeStr=uint8  RndMeth=Round
  Byte5（原回传字段4）_160 : DataTypeConversion  OutDataTypeStr=uint8  RndMeth=Round
  Byte6（原回传字段5）_161 : DataTypeConversion  OutDataTypeStr=uint8  RndMeth=Round
  Byte7（原回传字段6）_162 : DataTypeConversion  OutDataTypeStr=uint8  RndMeth=Round
  Byte8（原回传字段7）_163 : DataTypeConversion  OutDataTypeStr=uint8  RndMeth=Round
  Byte9（原回传字段8）_164 : DataTypeConversion  OutDataTypeStr=uint8  RndMeth=Round
  Constant（常量）_185 : Constant  Value=23  OutDataTypeStr=uint32
  Constant（常量）_187 : Constant  Value=27  OutDataTypeStr=uint32
  Constant（常量）_189 : Constant  Value=28  OutDataTypeStr=uint32
  Constant（常量）_192 : Constant  Value=0  OutDataTypeStr=uint8
  Counter23（第二十三字节填帧号）_186 : Assignment  DiagnosticForDimensions=Warning  IndexOptions=Index vector (port)  Indices=1  OutputSizes=1
  Fields（原回传字段顺序）_157 : BusSelector  OutputSignals=senddata1,senddata3,senddata4,senddata5,senddata6,senddata7,senddata8,senddata9,senddata10,senddata11,senddata12,senddata13,senddata14,senddata15,senddata16,senddata17,senddata18,senddata19,senddata20,senddata21,senddata22,senddata23,senddata24,senddata25,senddata26,senddata27
  Header（帧头AA55及类型一）_158 : Constant  Value=[170;85;1]  OutDataTypeStr=uint8
  High27（第二十七字节填泵速高字节）_188 : Assignment  DiagnosticForDimensions=Warning  IndexOptions=Index vector (port)  Indices=1  OutputSizes=1
  Low28（第二十八字节填泵速低字节）_190 : Assignment  DiagnosticForDimensions=Warning  IndexOptions=Index vector (port)  Indices=1  OutputSizes=1
  Original28（原二十八字节映射）_184 : Mux  Inputs=26
  SendEnabled（原回传开关非零）_193 : RelationalOperator  Operator=~=  OutDataTypeStr=boolean  RndMeth=Simplest  InputSameDT=off
  Payload（不含校验的二十八字节）_191 : Outport
  Enabled（上位机回传开关有效）_194 : Outport  Port=2
  wires:
  SendEnabled（原回传开关非零）_193/1 -> Enabled（上位机回传开关有效）_194/1  "SendEnabled（原回传开关非零）"
  Constant（常量）_192/1 -> SendEnabled（原回传开关非零）_193/2  "Constant（常量）"
  Fields（原回传字段顺序）_157/1 -> SendEnabled（原回传开关非零）_193/1  "<senddata1>"
  Low28（第二十八字节填泵速低字节）_190/1 -> Payload（不含校验的二十八字节）_191/1  "Low28（第二十八字节填泵速低字节）"
  Constant（常量）_189/1 -> Low28（第二十八字节填泵速低字节）_190/3  "Constant（常量）"
  Low（泵速低字节）_156/1 -> Low28（第二十八字节填泵速低字节）_190/2  "Low（泵速低字节）"
  High27（第二十七字节填泵速高字节）_188/1 -> Low28（第二十八字节填泵速低字节）_190/1  "High27（第二十七字节填泵速高字节）"
  Constant（常量）_187/1 -> High27（第二十七字节填泵速高字节）_188/3  "Constant（常量）"
  High（泵速高字节）_155/1 -> High27（第二十七字节填泵速高字节）_188/2  "High（泵速高字节）"
  Counter23（第二十三字节填帧号）_186/1 -> High27（第二十七字节填泵速高字节）_188/1  "Counter23（第二十三字节填帧号）"
  Constant（常量）_185/1 -> Counter23（第二十三字节填帧号）_186/3  "Constant（常量）"
  Counter（本帧帧号）_154/1 -> Counter23（第二十三字节填帧号）_186/2  "Counter（本帧帧号）"
  Original28（原二十八字节映射）_184/1 -> Counter23（第二十三字节填帧号）_186/1  "Original28（原二十八字节映射）"
  Byte28（原回传字段27）_183/1 -> Original28（原二十八字节映射）_184/26  "Byte28（原回传字段27）"
  Byte27（原回传字段26）_182/1 -> Original28（原二十八字节映射）_184/25  "Byte27（原回传字段26）"
  Byte26（原回传字段25）_181/1 -> Original28（原二十八字节映射）_184/24  "Byte26（原回传字段25）"
  Byte25（原回传字段24）_180/1 -> Original28（原二十八字节映射）_184/23  "Byte25（原回传字段24）"
  Byte24（原回传字段23）_179/1 -> Original28（原二十八字节映射）_184/22  "Byte24（原回传字段23）"
  Byte23（原回传字段22）_178/1 -> Original28（原二十八字节映射）_184/21  "Byte23（原回传字段22）"
  Byte22（原回传字段21）_177/1 -> Original28（原二十八字节映射）_184/20  "Byte22（原回传字段21）"
  Byte21（原回传字段20）_176/1 -> Original28（原二十八字节映射）_184/19  "Byte21（原回传字段20）"
  Byte20（原回传字段19）_175/1 -> Original28（原二十八字节映射）_184/18  "Byte20（原回传字段19）"
  Byte19（原回传字段18）_174/1 -> Original28（原二十八字节映射）_184/17  "Byte19（原回传字段18）"
  Byte18（原回传字段17）_173/1 -> Original28（原二十八字节映射）_184/16  "Byte18（原回传字段17）"
  Byte17（原回传字段16）_172/1 -> Original28（原二十八字节映射）_184/15  "Byte17（原回传字段16）"
  Byte16（原回传字段15）_171/1 -> Original28（原二十八字节映射）_184/14  "Byte16（原回传字段15）"
  Byte15（原回传字段14）_170/1 -> Original28（原二十八字节映射）_184/13  "Byte15（原回传字段14）"
  Byte14（原回传字段13）_169/1 -> Original28（原二十八字节映射）_184/12  "Byte14（原回传字段13）"
  Byte13（原回传字段12）_168/1 -> Original28（原二十八字节映射）_184/11  "Byte13（原回传字段12）"
  Byte12（原回传字段11）_167/1 -> Original28（原二十八字节映射）_184/10  "Byte12（原回传字段11）"
  Byte11（原回传字段10）_166/1 -> Original28（原二十八字节映射）_184/9  "Byte11（原回传字段10）"
  Byte10（原回传字段9）_165/1 -> Original28（原二十八字节映射）_184/8  "Byte10（原回传字段9）"
  Byte9（原回传字段8）_164/1 -> Original28（原二十八字节映射）_184/7  "Byte9（原回传字段8）"
  Byte8（原回传字段7）_163/1 -> Original28（原二十八字节映射）_184/6  "Byte8（原回传字段7）"
  Byte7（原回传字段6）_162/1 -> Original28（原二十八字节映射）_184/5  "Byte7（原回传字段6）"
  Byte6（原回传字段5）_161/1 -> Original28（原二十八字节映射）_184/4  "Byte6（原回传字段5）"
  Byte5（原回传字段4）_160/1 -> Original28（原二十八字节映射）_184/3  "Byte5（原回传字段4）"
  Byte4（原回传字段3）_159/1 -> Original28（原二十八字节映射）_184/2  "Byte4（原回传字段3）"
  Header（帧头AA55及类型一）_158/1 -> Original28（原二十八字节映射）_184/1  "Header（帧头AA55及类型一）"
  Fields（原回传字段顺序）_157/26 -> Byte28（原回传字段27）_183/1  "<senddata27>"
  Fields（原回传字段顺序）_157/25 -> Byte27（原回传字段26）_182/1  "<senddata26>"
  Fields（原回传字段顺序）_157/24 -> Byte26（原回传字段25）_181/1  "<senddata25>"
  Fields（原回传字段顺序）_157/23 -> Byte25（原回传字段24）_180/1  "<senddata24>"
  Fields（原回传字段顺序）_157/22 -> Byte24（原回传字段23）_179/1  "<senddata23>"
  Fields（原回传字段顺序）_157/21 -> Byte23（原回传字段22）_178/1  "<senddata22>"
  Fields（原回传字段顺序）_157/20 -> Byte22（原回传字段21）_177/1  "<senddata21>"
  Fields（原回传字段顺序）_157/19 -> Byte21（原回传字段20）_176/1  "<senddata20>"
  Fields（原回传字段顺序）_157/18 -> Byte20（原回传字段19）_175/1  "<senddata19>"
  Fields（原回传字段顺序）_157/17 -> Byte19（原回传字段18）_174/1  "<senddata18>"
  Fields（原回传字段顺序）_157/16 -> Byte18（原回传字段17）_173/1  "<senddata17>"
  Fields（原回传字段顺序）_157/15 -> Byte17（原回传字段16）_172/1  "<senddata16>"
  Fields（原回传字段顺序）_157/14 -> Byte16（原回传字段15）_171/1  "<senddata15>"
  Fields（原回传字段顺序）_157/13 -> Byte15（原回传字段14）_170/1  "<senddata14>"
  Fields（原回传字段顺序）_157/12 -> Byte14（原回传字段13）_169/1  "<senddata13>"
  Fields（原回传字段顺序）_157/11 -> Byte13（原回传字段12）_168/1  "<senddata12>"
  Fields（原回传字段顺序）_157/10 -> Byte12（原回传字段11）_167/1  "<senddata11>"
  Fields（原回传字段顺序）_157/9 -> Byte11（原回传字段10）_166/1  "<senddata10>"
  Fields（原回传字段顺序）_157/8 -> Byte10（原回传字段9）_165/1  "<senddata9>"
  Fields（原回传字段顺序）_157/7 -> Byte9（原回传字段8）_164/1  "<senddata8>"
  Fields（原回传字段顺序）_157/6 -> Byte8（原回传字段7）_163/1  "<senddata7>"
  Fields（原回传字段顺序）_157/5 -> Byte7（原回传字段6）_162/1  "<senddata6>"
  Fields（原回传字段顺序）_157/4 -> Byte6（原回传字段5）_161/1  "<senddata5>"
  Fields（原回传字段顺序）_157/3 -> Byte5（原回传字段4）_160/1  "<senddata4>"
  Fields（原回传字段顺序）_157/2 -> Byte4（原回传字段3）_159/1  "<senddata3>"
  Send（原回传字段总线）_153/1 -> Fields（原回传字段顺序）_157/1  "Send（原回传字段总线）"

== system turbo_controller/BoardOutput_串口封装与阀门时序/Out03_Telemetry（上位机回传组帧）/PumpBytes（泵速转高低字节）_152 ==
  note: 把泵速拆成高字节和低字节
      |
      | 输入来自Out01_Pump的平滑反馈泵速，可能仍有小数。先按本页既有取整和uint16转换规则得到16位值
      | U，再拆成两个可放进协议帧的字节：
      | 高字节 = floor(U/256)；
      | 低字节 = bitand(U,255)。
      |
      | 例如U=1000，高字节为3、低字节为232，因为3×256+232=1000。上位机必须把两个字节按同样顺序合起
      | 来，不能把232单独当成完整泵速。
      |
      | High和Low交给Payload，分别覆盖第27和28字节。这里只有数据编码，不再低通滤波，也没有修改油泵
      | 给定命令。
  Pump（滤波后的油泵转速）_139 : Inport  OutDataTypeStr=single
  Cast（数据类型转换）_142 : DataTypeConversion  OutDataTypeStr=double  RndMeth=Round
  Constant（常量）_143 : Constant  Value=256  OutDataTypeStr=double
  Constant（常量）_147 : Constant  Value=255  OutDataTypeStr=uint16
  Divide（相除）_144 : Product  Inputs=*/  SaturateOnIntegerOverflow=on  OutDataTypeStr=Inherit: Same as first input
  HighByte（高八位）_146 : DataTypeConversion  OutDataTypeStr=uint8  RndMeth=Floor
  Limit（限制到十六位无符号范围）_140 : Saturate  UpperLimit=65535  LowerLimit=0
  LowByte（低八位）_149 : DataTypeConversion  OutDataTypeStr=uint8  RndMeth=Floor
  LowMask（取低八位）_148 : simulink/Logic and Bit Operations/Bitwise Operator  logicop=AND  UseBitMask=off  NumInputPorts=2  BitMask=bin2dec('11011001')  BitMaskRealWorld=Stored Integer
      settings: LibrarySourceBlock=|
      | hdlsllib/Logic and Bit
      | Operations/Bitwise
      | Operator
  Round（保持原四舍五入规则）_141 : DataTypeConversion  OutDataTypeStr=uint16  RndMeth=Round
  Round（取整）_145 : Rounding
  High（泵速高字节）_150 : Outport
  Low（泵速低字节）_151 : Outport  Port=2
  wires:
  LowByte（低八位）_149/1 -> Low（泵速低字节）_151/1  "LowByte（低八位）"
  HighByte（高八位）_146/1 -> High（泵速高字节）_150/1  "HighByte（高八位）"
  LowMask（取低八位）_148/1 -> LowByte（低八位）_149/1  "LowMask（取低八位）"
  Constant（常量）_147/1 -> LowMask（取低八位）_148/2  "Constant（常量）"
  Round（取整）_145/1 -> HighByte（高八位）_146/1  "Round（取整）"
  Divide（相除）_144/1 -> Round（取整）_145/1  "Divide（相除）"
  Constant（常量）_143/1 -> Divide（相除）_144/2  "Constant（常量）"
  Cast（数据类型转换）_142/1 -> Divide（相除）_144/1  "Cast（数据类型转换）"
  Round（保持原四舍五入规则）_141/1 -> LowMask（取低八位）_148/1, Cast（数据类型转换）_142/1  "Round（保持原四舍五入规则）"
  Limit（限制到十六位无符号范围）_140/1 -> Round（保持原四舍五入规则）_141/1  "Limit（限制到十六位无符号范围）"
  Pump（滤波后的油泵转速）_139/1 -> Limit（限制到十六位无符号范围）_140/1  "Pump（滤波后的油泵转速）"

== system turbo_controller/BoardOutput_串口封装与阀门时序/Out04_Command（电机及油泵指令）/MotorFrame（电机指令高字节固定为零）_925 ==
  note: 电机的两个命令字节怎样装成九字节帧
      |
      | 父级把高命令字节固定0，低命令字节来自电机给定。这里不重新决定给定大小，只把这两个字节包装
      | 为外设协议。
      |
      | 前五项固定为十六进制AA、55、03、00、02；第6、7项依次放命令高字节与低字节。CRC16只以第6、7
      | 两项为输入，计算出16位校验值，再把CRC高字节放第8项、低字节放第9项。
      |
      | 完整帧 = [AA;55;03;00;02;CmdH;CmdL;CRCH;CRCL]。
      | 例如命令高0、低100表示两字节数100；CRC必须用[0,100]按本工程CRC表算出，不能只校验100或把AA5
      | 5头部也算进去。
      |
      | 9项帧交给父级，由20 ms发送许可和长度控制是否实际发送；本模块本身不操作串口。
  HighByte（给定高字节）_877 : Inport
  LowByte（给定低字节）_879 : Inport  Port=2
  CRC16（只校验两个命令字节）_912 : Subsystem  Description=|
      | 整段字节如何逐个累积CRC16
      | 
      | 这里的输入Bytes是发给外设的两个命令字节，不含前五项帧头。CRC的作用是把整段字节压缩成一个16位检查值，便于接收方发现传输内容变化。
      | 
      | 每帧从初始CRC=uint16(0)开始。循环一次取一个字节，把该字节乘256移到高8位，与旧CRC异或，得到Merged，再交给TableStep执行查表移位。TableStep的输出成为处理下一个字节的旧CRC。
      | 
      | 公式第一步是Merged=bitxor(旧CRC,当前字节×256)。整个循环结束后输出最后一次CRC，父级拆成高、低字节用于比较或发送。For Iterator中的CRC记忆是帧内累积状态，不能理解成跨帧无限累加。
      | 
      | 这里用的是CRC16_Table_Reference指定的算法表，不能随意换另一种CRC表或初始值。相同字节、顺序、表和初值必须得到相同结果，双方才能校验通过。
  Cast（数据类型转换）_878 : DataTypeConversion  OutDataTypeStr=uint8  RndMeth=Round
  Cast（数据类型转换）_880 : DataTypeConversion  OutDataTypeStr=uint8  RndMeth=Round
  Cast（数据类型转换）_913 : DataTypeConversion  OutDataTypeStr=double  RndMeth=Round
  Command（两个命令字节）_881 : Mux  Inputs=2
  Constant（常量）_914 : Constant  Value=256  OutDataTypeStr=double
  Constant（常量）_918 : Constant  Value=255  OutDataTypeStr=uint16
  Divide（相除）_915 : Product  Inputs=*/  SaturateOnIntegerOverflow=on  OutDataTypeStr=Inherit: Same as first input
  Frame9（完整九字节外设指令）_922 : Mux  Inputs=5
  Header（帧头AA55类型三长度二）_921 : Constant  Value=[170;85;3;0;2]  OutDataTypeStr=uint8
  HighByte（高八位）_917 : DataTypeConversion  OutDataTypeStr=uint8  RndMeth=Floor
  LowByte（低八位）_920 : DataTypeConversion  OutDataTypeStr=uint8  RndMeth=Floor
  LowMask（取低八位）_919 : simulink/Logic and Bit Operations/Bitwise Operator  logicop=AND  UseBitMask=off  NumInputPorts=2  BitMask=bin2dec('11011001')  BitMaskRealWorld=Stored Integer
      settings: LibrarySourceBlock=|
      | hdlsllib/Logic and Bit
      | Operations/Bitwise
      | Operator
  Round（取整）_916 : Rounding
  Frame（含校验的完整指令帧）_923 : Outport
  wires:
  Frame9（完整九字节外设指令）_922/1 -> Frame（含校验的完整指令帧）_923/1  "Frame9（完整九字节外设指令）"
  LowByte（低八位）_920/1 -> Frame9（完整九字节外设指令）_922/5  "LowByte（低八位）"
  HighByte（高八位）_917/1 -> Frame9（完整九字节外设指令）_922/4  "HighByte（高八位）"
  Header（帧头AA55类型三长度二）_921/1 -> Frame9（完整九字节外设指令）_922/1  "Header（帧头AA55类型三长度二）"
  LowMask（取低八位）_919/1 -> LowByte（低八位）_920/1  "LowMask（取低八位）"
  Constant（常量）_918/1 -> LowMask（取低八位）_919/2  "Constant（常量）"
  Round（取整）_916/1 -> HighByte（高八位）_917/1  "Round（取整）"
  Divide（相除）_915/1 -> Round（取整）_916/1  "Divide（相除）"
  Constant（常量）_914/1 -> Divide（相除）_915/2  "Constant（常量）"
  Cast（数据类型转换）_913/1 -> Divide（相除）_915/1  "Cast（数据类型转换）"
  CRC16（只校验两个命令字节）_912/1(CRC16（本帧校验结果）_911) -> Cast（数据类型转换）_913/1, LowMask（取低八位）_919/1  "CRC16（只校验两个命令字节）"
  Command（两个命令字节）_881/1 -> CRC16（只校验两个命令字节）_912/1(Bytes（待校验字节）_882)  "Command（两个命令字节）"
  Cast（数据类型转换）_880/1 -> Command（两个命令字节）_881/2, Frame9（完整九字节外设指令）_922/3  "Cast（数据类型转换）"
  Cast（数据类型转换）_878/1 -> Command（两个命令字节）_881/1, Frame9（完整九字节外设指令）_922/2  "Cast（数据类型转换）"
  LowByte（给定低字节）_879/1 -> Cast（数据类型转换）_880/1  "LowByte（给定低字节）"
  HighByte（给定高字节）_877/1 -> Cast（数据类型转换）_878/1  "HighByte（给定高字节）"

== system turbo_controller/BoardOutput_串口封装与阀门时序/Out04_Command（电机及油泵指令）/PumpFrame（油泵指令使用原高低给定字节）_973 ==
  note: 油泵的两个命令字节怎样装成九字节帧
      |
      | 父级传入原油泵给定的高、低两个命令字节。这里不重新决定给定大小，只把这两个字节包装为外设协
      | 议。
      |
      | 前五项固定为十六进制AA、55、03、00、02；第6、7项依次放命令高字节与低字节。CRC16只以第6、7
      | 两项为输入，计算出16位校验值，再把CRC高字节放第8项、低字节放第9项。
      |
      | 完整帧 = [AA;55;03;00;02;CmdH;CmdL;CRCH;CRCL]。
      | 例如命令高0、低100表示两字节数100；CRC必须用[0,100]按本工程CRC表算出，不能只校验100或把AA5
      | 5头部也算进去。
      |
      | 9项帧交给父级，由20 ms发送许可和长度控制是否实际发送；本模块本身不操作串口。
  HighByte（给定高字节）_926 : Inport
  LowByte（给定低字节）_928 : Inport  Port=2
  CRC16（只校验两个命令字节）_961 : Subsystem  Description=|
      | 整段字节如何逐个累积CRC16
      | 
      | 这里的输入Bytes是发给外设的两个命令字节，不含前五项帧头。CRC的作用是把整段字节压缩成一个16位检查值，便于接收方发现传输内容变化。
      | 
      | 每帧从初始CRC=uint16(0)开始。循环一次取一个字节，把该字节乘256移到高8位，与旧CRC异或，得到Merged，再交给TableStep执行查表移位。TableStep的输出成为处理下一个字节的旧CRC。
      | 
      | 公式第一步是Merged=bitxor(旧CRC,当前字节×256)。整个循环结束后输出最后一次CRC，父级拆成高、低字节用于比较或发送。For Iterator中的CRC记忆是帧内累积状态，不能理解成跨帧无限累加。
      | 
      | 这里用的是CRC16_Table_Reference指定的算法表，不能随意换另一种CRC表或初始值。相同字节、顺序、表和初值必须得到相同结果，双方才能校验通过。
  Cast（数据类型转换）_927 : DataTypeConversion  OutDataTypeStr=uint8  RndMeth=Round
  Cast（数据类型转换）_929 : DataTypeConversion  OutDataTypeStr=uint8  RndMeth=Round
  Cast（数据类型转换）_962 : DataTypeConversion  OutDataTypeStr=double  RndMeth=Round
  Command（两个命令字节）_930 : Mux  Inputs=2
  Constant（常量）_963 : Constant  Value=256  OutDataTypeStr=double
  Constant（常量）_967 : Constant  Value=255  OutDataTypeStr=uint16
  Divide（相除）_964 : Product  Inputs=*/  SaturateOnIntegerOverflow=on  OutDataTypeStr=Inherit: Same as first input
  Frame9（完整九字节外设指令）_971 : Mux  Inputs=5
  Header（帧头AA55类型三长度二）_970 : Constant  Value=[170;85;3;0;2]  OutDataTypeStr=uint8
  HighByte（高八位）_966 : DataTypeConversion  OutDataTypeStr=uint8  RndMeth=Floor
  LowByte（低八位）_969 : DataTypeConversion  OutDataTypeStr=uint8  RndMeth=Floor
  LowMask（取低八位）_968 : simulink/Logic and Bit Operations/Bitwise Operator  logicop=AND  UseBitMask=off  NumInputPorts=2  BitMask=bin2dec('11011001')  BitMaskRealWorld=Stored Integer
      settings: LibrarySourceBlock=|
      | hdlsllib/Logic and Bit
      | Operations/Bitwise
      | Operator
  Round（取整）_965 : Rounding
  Frame（含校验的完整指令帧）_972 : Outport
  wires:
  Frame9（完整九字节外设指令）_971/1 -> Frame（含校验的完整指令帧）_972/1  "Frame9（完整九字节外设指令）"
  LowByte（低八位）_969/1 -> Frame9（完整九字节外设指令）_971/5  "LowByte（低八位）"
  HighByte（高八位）_966/1 -> Frame9（完整九字节外设指令）_971/4  "HighByte（高八位）"
  Header（帧头AA55类型三长度二）_970/1 -> Frame9（完整九字节外设指令）_971/1  "Header（帧头AA55类型三长度二）"
  LowMask（取低八位）_968/1 -> LowByte（低八位）_969/1  "LowMask（取低八位）"
  Constant（常量）_967/1 -> LowMask（取低八位）_968/2  "Constant（常量）"
  Round（取整）_965/1 -> HighByte（高八位）_966/1  "Round（取整）"
  Divide（相除）_964/1 -> Round（取整）_965/1  "Divide（相除）"
  Constant（常量）_963/1 -> Divide（相除）_964/2  "Constant（常量）"
  Cast（数据类型转换）_962/1 -> Divide（相除）_964/1  "Cast（数据类型转换）"
  CRC16（只校验两个命令字节）_961/1(CRC16（本帧校验结果）_960) -> Cast（数据类型转换）_962/1, LowMask（取低八位）_968/1  "CRC16（只校验两个命令字节）"
  Command（两个命令字节）_930/1 -> CRC16（只校验两个命令字节）_961/1(Bytes（待校验字节）_931)  "Command（两个命令字节）"
  Cast（数据类型转换）_929/1 -> Frame9（完整九字节外设指令）_971/3, Command（两个命令字节）_930/2  "Cast（数据类型转换）"
  Cast（数据类型转换）_927/1 -> Command（两个命令字节）_930/1, Frame9（完整九字节外设指令）_971/2  "Cast（数据类型转换）"
  LowByte（给定低字节）_928/1 -> Cast（数据类型转换）_929/1  "LowByte（给定低字节）"
  HighByte（给定高字节）_926/1 -> Cast（数据类型转换）_927/1  "HighByte（给定高字节）"

== system turbo_controller/BoardOutput_串口封装与阀门时序/Out05_Handoff（输出交接与软件复位）/ResetService（ST官方软件复位服务） ==
  note: 什么时候调用STM32软件复位
      |
      | 父级把非零复位请求转换成0或1次执行许可。这里用这个次数决定本次是否进入ExecutionMode：0次完
      | 全不调用，1次才执行对应运行方式的实现。
      |
      | 普通计算机仿真采用Simulation分支，该分支为空，不尝试复位电脑。生成目标代码采用Target分支，
      | 用官方C Caller调用CMSIS的NVIC_SystemReset，让STM32重新进入启动流程。
      |
      | 这里不是清零一个控制变量，而是最终硬件复位服务。要保存运行状态，应在复位前由上层FRAM事务完
      | 成对应保存；本模块不负责CRC、写入验证或恢复记录选择。
  Request（复位请求零或一）_1545 : Inport  OutDataTypeStr=uint32
  ExecutionMode（仿真与目标运行方式）_1550 : Subsystem  Description=|  Variant=on  VariantControlMode=sim codegen switching
      | 同一复位请求怎样区分电脑仿真与目标代码
      | 
      | 父级ResetService已经决定这次是否执行复位；本模块只负责选择运行方式对应的实现，而不是再判断温度、油门或指令。
      | 
      | Simulation是普通仿真分支，内部有意为空，因此可以在电脑运行控制模型而不执行STM32专用复位调用。
      | Target是目标代码分支，内部官方C Caller执行NVIC_SystemReset，作用于真正的控制器。
      | 
      | 两条分支是运行方式选择，不应当同时作为两个控制过程解释。进入某分支不代表FRAM已经保存成功，保存事务属于另一个模块。
  IfRequested（有复位请求才执行一次）_1546 : ForIterator  IterationSource=external  ShowIterationPort=off
  wires:
  Request（复位请求零或一）_1545/1 -> IfRequested（有复位请求才执行一次）_1546/1  "Request（复位请求零或一）"

== system turbo_controller/CLM/ClpControl/Aim__Parameter_Calculate ==
  note: 闭环计算之前要准备哪些参数
      |
      | 本层把反馈转速和上位机装订需求整理成一套控制参数，供CtrlLaw直接使用，不在这里计算最终油泵
      | 给定。
      |
      | Aim_AccMaxMin_Cal1先用进入闭环时的反馈值作为起点，对装订需求作上升/下降限制，得到目标Nc_de
      | m；目标不低于40000，当前给定下限为700、上限为8000。
      | PIParameter_Cal分别按实际转速与目标转速查表，获得两套Kp/Ki候选，再各取较小值作为本次系数。
      | 允许转速误差固定为300。
      |
      | 结果按字段打包为允许误差、目标转速、油泵下限、油泵上限、Kp、Ki六项。例如装订从40000升到500
      | 00，实际控制目标不会直接跳50000，而先经HoldFirst逐次逼近；系数也随目标/反馈工作点变化。
      |
      | 这些字段送同级CtrlLaw和Fault_Process。总线打包只是交接参数，不能把它理解成又积分一次或又滤
      | 波一次。
  S_Nc_Filter : Inport
      settings: AttributesFormatString=S_Nc_Filter（滤波后的转速）
  S_Dem_SpeedLoad : Inport  Port=2
      settings: AttributesFormatString=S_Dem_SpeedLoad（装订目标转速）
  Aim_AccMaxMin_Cal1 : Subsystem  Description=|
      | 把装订转速变成平缓变化的闭环目标
      | 
      | 输入一项是上位机装订需求，另一项是反馈转速。本模块先让HoldFirst锁住进入闭环时的有效转速，M_Rate_Limiter从这个起点逐次逼近装订值，再把目标与40000取较大值。
      | 
      | 所以Nc_dem=max(变化限制后的需求,40000)。例如需求低于40000，即使限速结果更低，送控制律的目标仍是40000。这是当前模型设置，不能把上位机原始需求直接当闭环最终目标。
      | 
      | 同时给出油泵给定下限700和上限8000。它们是本工程给定量的数值边界，不是转速上下限。后面的控制律和输出仲裁分别使用这些边界。
      | 
      | 输出Nc_dem送PI系数计算和误差计算；Acc_Min/Acc_Max送给定限幅和故障备用控制。这里没有直接改写实际测量转速。
      settings: AttributesFormatString=Aim_AccMaxMin_Cal1（目标油门上限下限计算1）
  Bus Creator1 : BusCreator  Inputs=6
      settings: AttributesFormatString=Bus Creator1（总线创建器1）
  Constant3 : Constant  Value=300  OutDataTypeStr=single
      settings: AttributesFormatString=Constant3（常量3）
  PIParameter_Cal : Subsystem  Description=|
      | Kp和Ki为什么要查两遍表
      | 
      | 闭环工作点会变化，同一个固定PI系数不一定适合全部转速。这里接收实际滤波转速和当前受限目标转速，对两者分别查Kp表与Ki表，共四次查表。
      | 
      | 两个Kp候选取较小值，两个Ki候选也取较小值，再乘当前统一增益1：
      | Kp=min(Kp表(反馈转速),Kp表(目标转速))；
      | Ki=min(Ki表(反馈转速),Ki表(目标转速))。
      | 
      | 断点覆盖约20654～60355 r/min，表中不同区段采用不同增益，断点之间按各查表块配置插值。例如某路候选Kp为0.02、另一路0.03，最终采用0.02，不把它们相加或平均。
      | 
      | Kp用于误差变化量的比例项，Ki用于当前误差项。这里仅准备参数，实际增量PI在CtrlLaw执行；也不能把Ki表值单独解释成已经乘过任意新增采样时间的连续积分系数。
      settings: AttributesFormatString=PIParameter_Cal（圆周率参数计算）
  S_Control_Parameter : Outport
      settings: AttributesFormatString=S_Control_Parameter（控制参数）
  wires:
  S_Nc_Filter/1 -> Aim_AccMaxMin_Cal1/2(S_Nc_Filter), PIParameter_Cal/1(S_Nc_Filter)
  Aim_AccMaxMin_Cal1/1(Nc_dem) -> Bus Creator1/2, PIParameter_Cal/2(S_Nc_dem)  "Nc_dem（控制目标转速）"
  Aim_AccMaxMin_Cal1/2(Acc_Min) -> Bus Creator1/3  "Acc_Min（油泵给定下限）"
  Aim_AccMaxMin_Cal1/3(Acc_Max) -> Bus Creator1/4  "Acc_Max（油泵给定上限）"
  PIParameter_Cal/1(Kp) -> Bus Creator1/5  "Kp（比例增益）"
  PIParameter_Cal/2(Ki) -> Bus Creator1/6  "Ki（积分增益）"
  Constant3/1 -> Bus Creator1/1  "RotaSpeed_ErrorAllow（转速允许偏差）"
  S_Dem_SpeedLoad/1 -> Aim_AccMaxMin_Cal1/1(S_Dem_SpeedLoad)
  Bus Creator1/1 -> S_Control_Parameter/1
